simulink model "Part2_2024b"  (R2024b)
settings: Solver=FixedStepAuto  StartTime=0.0  StopTime=20  FixedStep=Ts/100  RelTol=1e-3
values from neighbouring files (symbols this model uses):
  A_full = [   0,                           1,                         0,       0 ... (first row only)    [Part1_Part2_script.m]
  B_full = [           0,               0 ... (first row only)    [Part1_Part2_script.m]
  C_speed = minreal( (1/Gz_motor) * (F_star / (1 - F_star)) )    [Part1_Part2_script.m]
  Kp = 0.77    [Part1_Part2_script.m]
  nbit = 8    [Part1_Part2_script.m]
  wfilter_position = 20 * omega_c_pos_actual    [Part1_Part2_script.m]
  wfilter_speed = 27    [Part1_Part2_script.m]
undefined symbols (not defined in the file or in its folder): dspblkCoreblockFVToolHelper, gcbh
settings Model: Creator=karimdoubie  LastModifiedBy=Riccardo

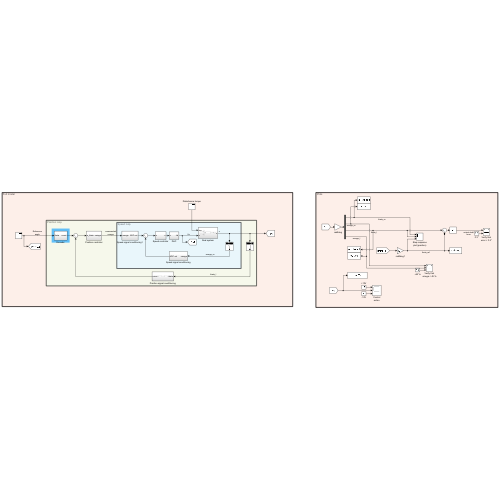
[thumbnail: Simulink's stored preview of the top-level diagram]
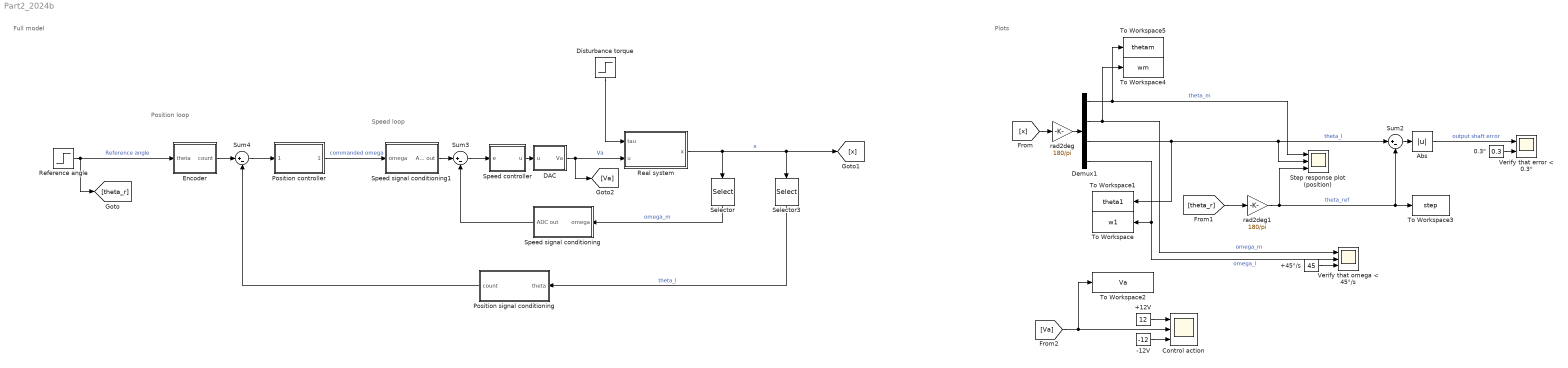
== system Part2_2024b ==
  note: Plots
  note: Position loop
  note: Speed loop
  note: Full model
  +12V : Constant  Value=12
  +45°/s : Constant  Value=45
  -12V : Constant  Value=-12
  0.3° : Constant  Value=0.3
  Abs : Abs  SaturateOnIntegerOverflow=off
  Control action : Scope  NumInputPorts=3
  DAC : Subsystem
  Demux1 : Demux
  Disturbance torque : Step  Time=6  After=0.05  SampleTime=0
  Encoder : Subsystem
  Position controller : Subsystem
  Position signal conditioning : Subsystem
  Real system : Subsystem
  Reference angle : Step  After=deg2rad(60)  SampleTime=0
  Selector : Selector  InputPortWidth=4  IndexOptions=Index vector (dialog)  Indices=2  OutputSizes=1
  Selector3 : Selector  InputPortWidth=4  IndexOptions=Index vector (dialog)  Indices=3  OutputSizes=1
  Speed controller : Subsystem
  Speed signal conditioning : Subsystem
  Speed signal conditioning1 : Subsystem
  Step response plot (position) : Scope  NumInputPorts=3
  Sum2 : Sum  Inputs=|+-
  Sum3 : Sum  Inputs=|+-
  Sum4 : Sum  Inputs=|+-
  To Workspace : ToWorkspace  VariableName=w1  SaveFormat=Timeseries  SampleTime=-1
  To Workspace1 : ToWorkspace  VariableName=theta1  SaveFormat=Timeseries  SampleTime=-1
  To Workspace2 : ToWorkspace  VariableName=Va  SaveFormat=Timeseries  SampleTime=-1
  To Workspace3 : ToWorkspace  VariableName=step  SaveFormat=Timeseries  SampleTime=-1
  To Workspace4 : ToWorkspace  VariableName=wm  SaveFormat=Timeseries  SampleTime=-1
  To Workspace5 : ToWorkspace  VariableName=thetam  SaveFormat=Timeseries  SampleTime=-1
  Verify that error < 0.3° : Scope  NumInputPorts=2
  Verify that omega < 45°/s : Scope  NumInputPorts=3
  rad2deg : Gain  Gain=180/pi
  rad2deg1 : Gain  Gain=180/pi
  wires:
  Position controller/1(omega) -> Speed signal conditioning1/1(omega)  "commanded omega"
  0.3°/1 -> Verify that error < 0.3°/2
  [theta_r] -> rad2deg1/1
  Demux1/1 -> To Workspace5/1, Step response plot (position)/1  "theta_m"
  rad2deg1/1 -> Step response plot (position)/3, To Workspace3/1, Sum2/2  "theta_ref"
  Demux1/2 -> To Workspace4/1, Verify that omega < 45°/s/1  "omega_m"
  Position signal conditioning/1(count) -> Sum4/2
  Speed controller/1(u) -> DAC/1(u)
  Demux1/4 -> Verify that omega < 45°/s/2, To Workspace/1  "omega_l"
  Demux1/3 -> Sum2/1, Step response plot (position)/2, To Workspace1/1  "theta_l"
  +45°/s/1 -> Verify that omega < 45°/s/3
  Reference angle/1 -> Encoder/1(theta), [theta_r]  "Reference angle"
  DAC/1(Va) -> [Va], Real system/2(u)  "Va"
  [x] -> rad2deg/1
  Real system/1(x) -> [x], Selector3/1, Selector/1  "x"
  Selector/1 -> Speed signal conditioning/1(omega)  "omega_m"
  Selector3/1 -> Position signal conditioning/1(theta)  "theta_l"
  Sum2/1 -> Abs/1
  Sum3/1 -> Speed controller/1(e)
  Speed signal conditioning1/1(ADC out) -> Sum3/1
  Sum4/1 -> Position controller/1(e_theta)
  Abs/1 -> Verify that error < 0.3°/1  "output shaft error"
  +12V/1 -> Control action/1
  -12V/1 -> Control action/3
  rad2deg/1 -> Demux1/1
  [Va] -> Control action/2, To Workspace2/1
  Disturbance torque/1 -> Real system/1(tau)
  Speed signal conditioning/1(ADC out) -> Sum3/2
  Encoder/1(count) -> Sum4/1

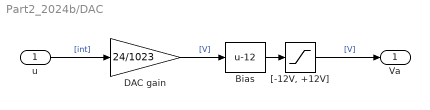
== system Part2_2024b/DAC ==
  u : Inport
  Bias : Bias  Bias=-12  SaturateOnIntegerOverflow=off
  DAC gain : Gain  Gain=24/1023
  "[-12V, +12V]" : Saturate  UpperLimit=12  LowerLimit=-12
  Va : Outport
  wires:
  "[-12V, +12V]"/1 -> Va/1  "[V]"
  Bias/1 -> "[-12V, +12V]"/1
  u/1 -> DAC gain/1  "[int]"
  DAC gain/1 -> Bias/1  "[V]"

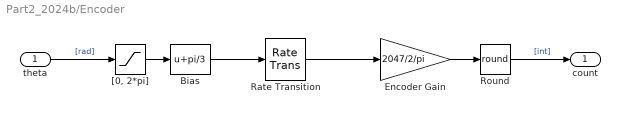
== system Part2_2024b/Encoder ==
  theta : Inport
  Bias : Bias  Bias=pi/3  SaturateOnIntegerOverflow=off
  Encoder Gain : Gain  Gain=2047/2/pi
  Rate Transition : RateTransition  OutPortSampleTime=Ts
  Round : Rounding  Operator=round
  "[0, 2*pi]" : Saturate  UpperLimit=2*pi  LowerLimit=0
  count : Outport
  wires:
  theta/1 -> "[0, 2*pi]"/1  "[rad]"
  Bias/1 -> Rate Transition/1
  Encoder Gain/1 -> Round/1
  Round/1 -> count/1  "[int]"
  "[0, 2*pi]"/1 -> Bias/1
  Rate Transition/1 -> Encoder Gain/1

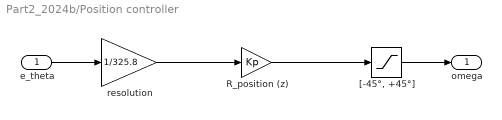
== system Part2_2024b/Position controller ==
  e_theta : Inport
  R_position (z) : Gain  Gain=Kp
  "[-45°, +45°]" : Saturate  UpperLimit=deg2rad(45)  LowerLimit=-deg2rad(45)
  resolution : Gain  Gain=1/325.8
  omega : Outport
  wires:
  e_theta/1 -> resolution/1
  R_position (z)/1 -> "[-45°, +45°]"/1
  resolution/1 -> R_position (z)/1
  "[-45°, +45°]"/1 -> omega/1

== system Part2_2024b/Position signal conditioning ==
  theta : Inport
  Encoder : Subsystem
  Lowpass filter (I order) : TransferFcn  Denominator=[1/wfilter_position 1]
  count : Outport
  wires:
  Lowpass filter (I order)/1 -> Encoder/1(theta)  "[rad/s]"
  theta/1 -> Lowpass filter (I order)/1  "[rad/s]"
  Encoder/1(count) -> count/1  "[int]"

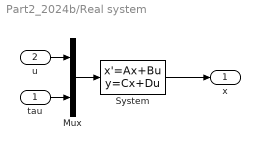
== system Part2_2024b/Real system ==
  tau : Inport
  u : Inport  Port=2
  Mux : Mux  Inputs=2
  System : StateSpace  A=A_full  B=B_full  C=eye(4)  D=[0 0 0 0; 0 0 0 0]'  InitialCondition=0
  x : Outport
  wires:
  tau/1 -> Mux/2
  Mux/1 -> System/1
  System/1 -> x/1
  u/1 -> Mux/1

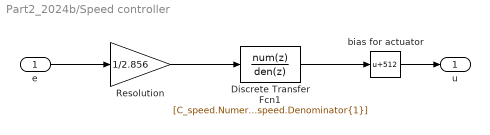
== system Part2_2024b/Speed controller ==
  e : Inport
  Discrete Transfer Fcn1 : DiscreteTransferFcn  LoadFcn=dspblkCoreblockFVToolHelper(gcbh,'load');  Numerator=[C_speed.Numerator{1}]  Denominator=[C_speed.Denominator{1}]
      settings: CopyFcn=dspblkCoreblockFVToolHelper(gcbh,'copy');  DeleteFcn=dspblkCoreblockFVToolHelper(gcbh,'close');  ModelCloseFcn=dspblkCoreblockFVToolHelper(gcbh,'close');  PreSaveFcn=dspblkCoreblockFVToolHelper(gcbh,'presave');  PostSaveFcn=dspblkCoreblockFVToolHelper(gcbh,'postsave');  CloseFcn=dspblkCoreblockFVToolHelper(gcbh,'close');
  Resolution : Gain  Gain=1/2.856
  bias for actuator : Bias  Bias=512  SaturateOnIntegerOverflow=off
  u : Outport
  wires:
  Discrete Transfer Fcn1/1 -> bias for actuator/1
  Resolution/1 -> Discrete Transfer Fcn1/1
  e/1 -> Resolution/1
  bias for actuator/1 -> u/1

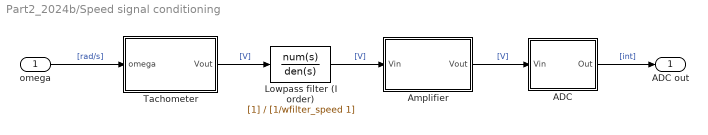
== system Part2_2024b/Speed signal conditioning ==
  omega : Inport
  ADC : Subsystem
  Amplifier : Subsystem
  Lowpass filter (I order) : TransferFcn  Denominator=[1/wfilter_speed 1]
  Tachometer : Subsystem
  ADC out : Outport
  wires:
  omega/1 -> Tachometer/1(omega)  "[rad/s]"
  ADC/1(Out) -> ADC out/1  "[int]"
  Tachometer/1(Vout) -> Lowpass filter (I order)/1  "[V]"
  Lowpass filter (I order)/1 -> Amplifier/1(Vin)  "[V]"
  Amplifier/1(Vout) -> ADC/1(Vin)  "[V]"

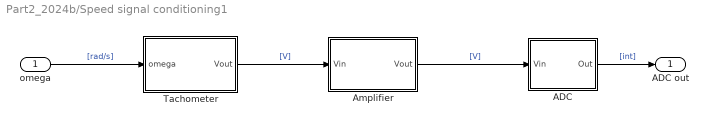
== system Part2_2024b/Speed signal conditioning1 ==
  omega : Inport
  ADC : Subsystem
  Amplifier : Subsystem
  Tachometer : Subsystem
  ADC out : Outport
  wires:
  omega/1 -> Tachometer/1(omega)  "[rad/s]"
  ADC/1(Out) -> ADC out/1  "[int]"
  Tachometer/1(Vout) -> Amplifier/1(Vin)  "[V]"
  Amplifier/1(Vout) -> ADC/1(Vin)  "[V]"

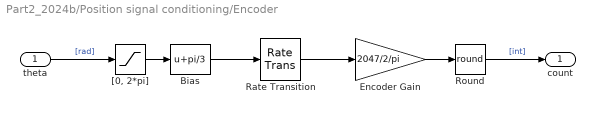
== system Part2_2024b/Position signal conditioning/Encoder ==
  theta : Inport
  Bias : Bias  Bias=pi/3  SaturateOnIntegerOverflow=off
  Encoder Gain : Gain  Gain=2047/2/pi
  Rate Transition : RateTransition  OutPortSampleTime=Ts
  Round : Rounding  Operator=round
  "[0, 2*pi]" : Saturate  UpperLimit=2*pi  LowerLimit=0
  count : Outport
  wires:
  theta/1 -> "[0, 2*pi]"/1  "[rad]"
  Bias/1 -> Rate Transition/1
  Encoder Gain/1 -> Round/1
  Round/1 -> count/1  "[int]"
  "[0, 2*pi]"/1 -> Bias/1
  Rate Transition/1 -> Encoder Gain/1

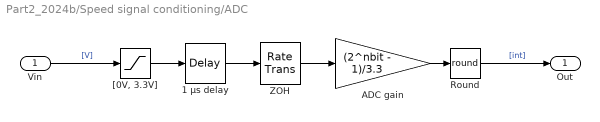
== system Part2_2024b/Speed signal conditioning/ADC ==
  Vin : Inport
  "1 µs delay " : TransportDelay  DelayTime=1e-6
  ADC gain : Gain  Gain=(2^nbit - 1)/3.3
  Round : Rounding  Operator=round
  ZOH : RateTransition  OutPortSampleTime=Ts
  "[0V, 3.3V] " : Saturate  UpperLimit=3.3  LowerLimit=0
  Out : Outport
  wires:
  Vin/1 -> "[0V, 3.3V] "/1  "[V]"
  ADC gain/1 -> Round/1
  ZOH/1 -> ADC gain/1
  Round/1 -> Out/1  "[int]"
  "[0V, 3.3V] "/1 -> "1 µs delay "/1
  "1 µs delay "/1 -> ZOH/1

== system Part2_2024b/Speed signal conditioning/Amplifier ==
  Vin : Inport
  a : Gain  Gain=2.75
  b : Bias  Bias=1.65  SaturateOnIntegerOverflow=off
  Vout : Outport
  wires:
  a/1 -> b/1
  b/1 -> Vout/1  "[V]"
  Vin/1 -> a/1  "[V]"

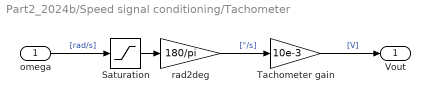
== system Part2_2024b/Speed signal conditioning/Tachometer ==
  omega : Inport
  Saturation : Saturate  UpperLimit=pi/3  LowerLimit=-pi/3
  Tachometer gain : Gain  Gain=10e-3
  rad2deg : Gain  Gain=180/pi
  Vout : Outport
  wires:
  omega/1 -> Saturation/1  "[rad/s]"
  rad2deg/1 -> Tachometer gain/1  "[°/s]"
  Tachometer gain/1 -> Vout/1  "[V]"
  Saturation/1 -> rad2deg/1

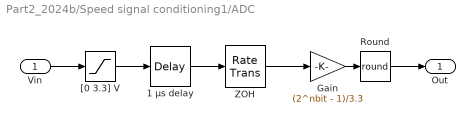
== system Part2_2024b/Speed signal conditioning1/ADC ==
  Vin : Inport
  "1 µs delay " : TransportDelay  DelayTime=1e-6
  Gain : Gain  Gain=(2^nbit - 1)/3.3
  Round : Rounding  Operator=round
  ZOH : RateTransition  OutPortSampleTime=Ts
  "[0 3.3] V" : Saturate  UpperLimit=3.3  LowerLimit=0
  Out : Outport
  wires:
  Vin/1 -> "[0 3.3] V"/1
  Gain/1 -> Round/1
  ZOH/1 -> Gain/1
  Round/1 -> Out/1
  "[0 3.3] V"/1 -> "1 µs delay "/1
  "1 µs delay "/1 -> ZOH/1

== system Part2_2024b/Speed signal conditioning1/Amplifier ==
  Vin : Inport
  Bias : Bias  Bias=3.3/2  SaturateOnIntegerOverflow=off
  Gain : Gain  Gain=3.3 / (2*0.6)
  Vout : Outport
  wires:
  Gain/1 -> Bias/1
  Bias/1 -> Vout/1  "[V]"
  Vin/1 -> Gain/1

== system Part2_2024b/Speed signal conditioning1/Tachometer ==
  omega : Inport
  Saturation : Saturate  UpperLimit=pi/3  LowerLimit=-pi/3
  Tachometer gain : Gain  Gain=10e-3
  rad2deg : Gain  Gain=180/pi
  Vout : Outport
  wires:
  omega/1 -> Saturation/1  "[rad/s]"
  rad2deg/1 -> Tachometer gain/1  "[°/s]"
  Tachometer gain/1 -> Vout/1  "[V]"
  Saturation/1 -> rad2deg/1
